simulink model "wturbines"  (R2024b)
settings: Solver=ode4  StartTime=0.0  StopTime=inf  FixedStep=0.01  RelTol=1e-3
values from neighbouring files (symbols this model uses):
  A_k = 2E6    (= 2000000)    [initialize_turbine_parameters.m]
  air_density = 1.225    [initialize_turbine_parameters.m]
  alpha_pitch_exp = 0    [initialize_turbine_parameters.m]
  B_k = 1E4    (= 10000)    [initialize_turbine_parameters.m]
  brake_torque = 28116.2    [initialize_turbine_parameters.m]
  C_k = 0    [initialize_turbine_parameters.m]
  Cp_mat = nan(numel(tsr_vec), numel(pitch_vec))    [initialize_turbine_parameters.m]
  Cp_opt = 0.482    [initialize_turbine_parameters.m]
  Ct_mat = nan(size(Cp_mat))    [initialize_turbine_parameters.m]
  ctrl_mode = 1    [initialize_turbine_parameters.m]
  cut_in_wind_speed = 3.0    (= 3)    [initialize_turbine_parameters.m]
  cut_out_wind_speed = 25.0    (= 25)    [initialize_turbine_parameters.m]
  D_k = 0    [initialize_turbine_parameters.m]
  dr_mode = Simulink.Parameter(1)    [initialize_turbine_parameters.m]
  gearbox_ratio = 1    [initialize_turbine_parameters.m]
  generator_eff = 0.954    [initialize_turbine_parameters.m]
  inertia = 1.9E6    (= 1900000)    [initialize_turbine_parameters.m]
  K_i_gen = 1e2    (= 100)    [initialize_turbine_parameters.m]
  K_i_pitch = 0    [initialize_turbine_parameters.m]
  K_i_pitch_gs = 0    [initialize_turbine_parameters.m]
  K_omega_sq = 1/2 * (tsr_opt)^-3 * air_density * pi * (rotor_diameter / 2)^5 * Cp_opt / gearbox_ratio^3    (= 69831977.2177)    [initialize_turbine_parameters.m]
  K_p_gen = 1e2    (= 100)    [initialize_turbine_parameters.m]
  K_p_pitch = 1    [initialize_turbine_parameters.m]
  K_p_pitch_gs = 0.1    [initialize_turbine_parameters.m]
  max_gen_torque = 1.15 * rated_gen_torque    (= 35686440.711)    [initialize_turbine_parameters.m]
  MIN_ROT_SPEED = 1e-3    (= 0.001)    [initialize_turbine_parameters.m]
  Nt = 9    [init.m]
  pitch_all = T{:, col_pitch}    [initialize_turbine_parameters.m]
  pitch_rate_deg = 5    [initialize_turbine_parameters.m]
  pitch_vec = sort(pitch_vec(:))    [initialize_turbine_parameters.m]
  rated_power = 22E6    (= 22000000)    [initialize_turbine_parameters.m]
  rated_rotor_speed = 6.77    [initialize_turbine_parameters.m]
  rated_rotor_speed_rads = rated_rotor_speed * (2 * pi) / 60    (= 0.70895274216)    [initialize_turbine_parameters.m]
  rated_wind_speed = 11.0    (= 11)    [initialize_turbine_parameters.m]
  ROT_EMG_MAX_TOL = 1.15    [initialize_turbine_parameters.m]
  ROT_SPEED_MIN_TRANS = min_rotor_speed_rads    (= 0.19)    [initialize_turbine_parameters.m]
  ROT_SPEED_SP_DIFF = 0.1    [initialize_turbine_parameters.m]
  rotor_radius = rotor_diameter / 2    (= 142)    [initialize_turbine_parameters.m]
  rotor_speed_all = [0, rated_rotor_speed]    [initialize_turbine_parameters.m]
  rotor_speed_init = rotor_speed_init * (2 * pi) / 60    (= 1.25663706144)    [initialize_turbine_parameters.m]
  rotor_speed_ref_mode = 1    [initialize_turbine_parameters.m]
  tsr_opt = 9.153    [initialize_turbine_parameters.m]
  tsr_vec = sort(tsr_vec(:))    [initialize_turbine_parameters.m]
  u_all = T{:, col_u}    [initialize_turbine_parameters.m]
  u_rotor_speed_all = [cut_in_wind_speed, rated_wind_speed]    [initialize_turbine_parameters.m]
  yawing_rate = 5    [initialize_turbine_parameters.m]
undefined symbols (not defined in the file or in its folder): op_mode, turbineDataBytes
libraries: simulink x24, simulink_extras x14, slpidlib x8, slrealtimeiplib x4, svdutilitieslib x2, slctrl_autotuning x2, etargetslib x2, dspstat3 x1
(part 1 of 3)
settings Model: SimulationMode=external  ExtModeEnableFloating=off  Creator=ivovanstraalen  LastModifiedBy=hackaton26
settings SolverCC: ConcurrentTasks=on  PositivePriorityOrder=on
settings DataIOCC: InspectSignalLogs=on
settings OptimizationCC: BlockReduction=off  OptimizeBlockIOStorage=off
settings DebuggingCC: SignalInfNanChecking=error  TasksWithSamePriorityMsg=none
settings HardwareCC: ProdBitPerLong=64  ProdLongLongMode=on  ProdHWDeviceType=Intel->x86-64 (Linux 64)
settings RTWCC: Description=Speedgoat Real-Time Target Machine  SystemTargetFile=speedgoat.tlc  TemplateMakefile=slrealtime_default_tmf  Toolchain=Simulink Real-Time Toolchain  BuildConfiguration=Faster Runs  CodeExecutionProfiling=on  TargetLang=C++
settings SimulinkRealTimeTargetCC: InstructionSetFMA=off  LogToMDFFile=off

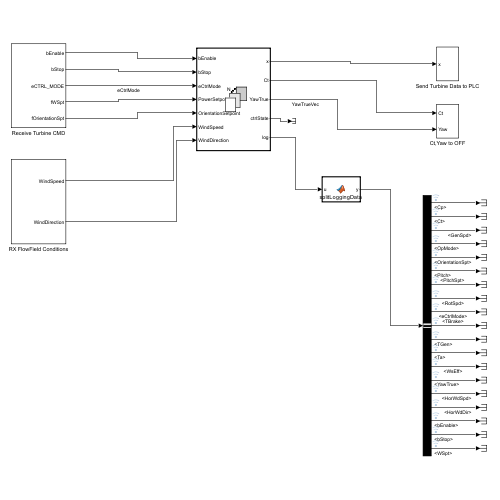
[thumbnail: Simulink's stored preview of the top-level diagram]
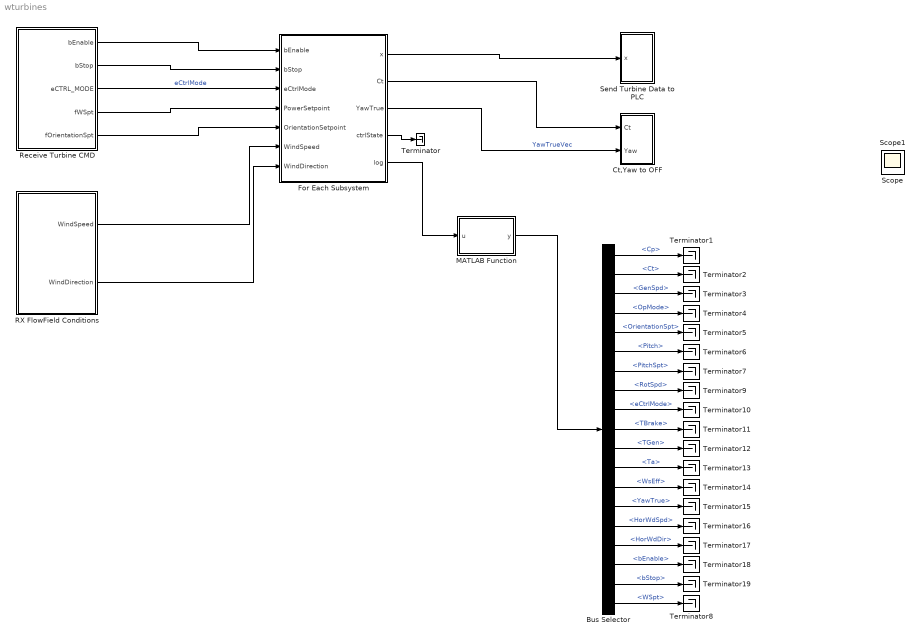
== system wturbines ==
  Bus Selector : BusSelector  OutputSignals=Cp,Ct,GenSpd,OpMode,OrientationSpt,Pitch,PitchSpt,RotSpd,eCtrlMode,TBrake,TGen,Ta,WsEff,YawTrue,HorWdSpd,HorWdDir,bEnable,bStop,WSpt
  Ct,Yaw to OFF : Subsystem
  For Each Subsystem : Subsystem  TreatAsAtomicUnit=on
  MATLAB Function : MATLAB Function  TreatAsAtomicUnit=on
  RX FlowField Conditions : Subsystem
  Receive Turbine CMD : Subsystem
  Send Turbine Data to PLC : Subsystem
  Terminator{,1..19} (20 alike) : Terminator
  Scope : Scope
  Scope1 : Scope
  wires:
  For Each Subsystem/1(x) -> Send Turbine Data to PLC/1(x)
  Receive Turbine CMD/1(bEnable) -> For Each Subsystem/1(bEnable)
  Receive Turbine CMD/4(fWSpt) -> For Each Subsystem/4(PowerSetpoint)
  Receive Turbine CMD/5(fOrientationSpt) -> For Each Subsystem/5(OrientationSetpoint)
  For Each Subsystem/2(Ct) -> Ct,Yaw to OFF/1(Ct)
  For Each Subsystem/3(YawTrue) -> Ct,Yaw to OFF/2(Yaw)  "YawTrueVec"
  RX FlowField Conditions/1(WindSpeed) -> For Each Subsystem/6(WindSpeed)
  RX FlowField Conditions/2(WindDirection) -> For Each Subsystem/7(WindDirection)
  Receive Turbine CMD/2(bStop) -> For Each Subsystem/2(bStop)
  Receive Turbine CMD/3(eCTRL_MODE) -> For Each Subsystem/3(eCtrlMode)  "eCtrlMode"
  For Each Subsystem/4(ctrlState) -> Terminator/1
  For Each Subsystem/5(log) -> MATLAB Function/1(u)
  MATLAB Function/1(y) -> Bus Selector/1
  Bus Selector/1 -> Terminator1/1  "<Cp>"
  Bus Selector/2 -> Terminator2/1  "<Ct>"
  Bus Selector/3 -> Terminator3/1  "<GenSpd>"
  Bus Selector/4 -> Terminator4/1  "<OpMode>"
  Bus Selector/5 -> Terminator5/1  "<OrientationSpt>"
  Bus Selector/6 -> Terminator6/1  "<Pitch>"
  Bus Selector/7 -> Terminator7/1  "<PitchSpt>"
  Bus Selector/8 -> Terminator9/1  "<RotSpd>"
  Bus Selector/9 -> Terminator10/1  "<eCtrlMode>"
  Bus Selector/10 -> Terminator11/1  "<TBrake>"
  Bus Selector/11 -> Terminator12/1  "<TGen>"
  Bus Selector/12 -> Terminator13/1  "<Ta>"
  Bus Selector/13 -> Terminator14/1  "<WsEff>"
  Bus Selector/14 -> Terminator15/1  "<YawTrue>"
  Bus Selector/15 -> Terminator16/1  "<HorWdSpd>"
  Bus Selector/16 -> Terminator17/1  "<HorWdDir>"
  Bus Selector/17 -> Terminator18/1  "<bEnable>"
  Bus Selector/18 -> Terminator19/1  "<bStop>"
  Bus Selector/19 -> Terminator8/1  "<WSpt>"

== system wturbines/Ct,Yaw to OFF ==
  Ct : Inport
  Yaw : Inport  Port=2
  Byte Pack1 : svdutilitieslib/Byte Pack  maskPackedDataType=uint8  datatypes={'single'}  byteAlign=1  blockPlatform=tic2000
      settings: LibrarySourceBlock=c2000lib/Target Communication/Byte Pack
  Constant1 : Constant  Value=Nt * 2*4
  Data Type Conversion : DataTypeConversion  OutDataTypeStr=single  SaturateOnIntegerOverflow=off  RndMeth=Floor
  Mux : Mux  Inputs=2
  Rate Transition : RateTransition
  UDP Send1 : slrealtimeiplib/UDP Send  useHostTargetConn=off  toAddress=pcIP  toPort=pcRXport  sampleTime=Ts_FF  enableMessage=off  ipAddress=localIP  localPort=rtsTXFFport
  wires:
  Data Type Conversion/1 -> Byte Pack1/1
  Constant1/1 -> UDP Send1/2
  Byte Pack1/1 -> UDP Send1/1
  Rate Transition/1 -> Data Type Conversion/1
  Yaw/1 -> Mux/2
  Ct/1 -> Mux/1
  Mux/1 -> Rate Transition/1

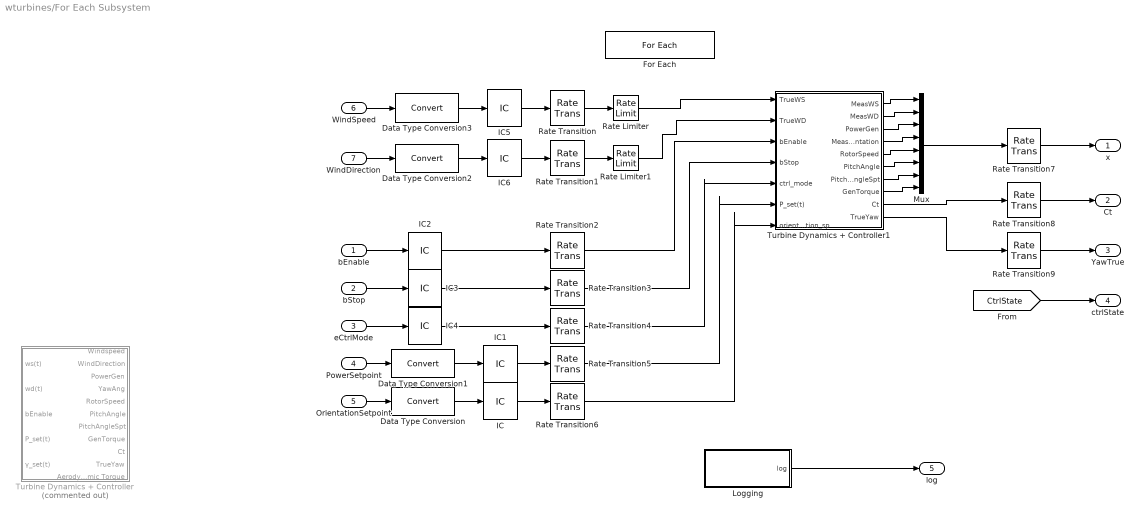
== system wturbines/For Each Subsystem ==
  bEnable : Inport  Partition=on  PartitionDimension=1  PartitionWidth=1  PartitionOffset=0
  bStop : Inport  Port=2  Partition=on  PartitionDimension=1  PartitionWidth=1  PartitionOffset=0
  eCtrlMode : Inport  Port=3  Partition=on  PartitionDimension=1  PartitionWidth=1  PartitionOffset=0
  PowerSetpoint : Inport  Port=4  Partition=on  PartitionDimension=1  PartitionWidth=1  PartitionOffset=0
  OrientationSetpoint : Inport  Port=5  Partition=on  PartitionDimension=1  PartitionWidth=1  PartitionOffset=0
  WindSpeed : Inport  Port=6  Partition=on  PartitionDimension=1  PartitionWidth=1  PartitionOffset=0
  WindDirection : Inport  Port=7  Partition=on  PartitionDimension=1  PartitionWidth=1  PartitionOffset=0
  Data Type Conversion{,1..3} (4 alike) : DataTypeConversion  SaturateOnIntegerOverflow=off  RndMeth=Floor
  For Each : ForEach  DisableCoverage=on  ShowIterationIndex=on
  IC : InitialCondition  Value=270
  IC1 : InitialCondition  Value=-1
  IC2 : InitialCondition  Value=false
  IC3 : InitialCondition  Value=false
  IC4 : InitialCondition
  IC5 : InitialCondition  Value=0
  IC6 : InitialCondition  Value=0
  Logging : Subsystem
  Mux : Mux  Inputs=8
  Rate Limiter : RateLimiter  RisingSlewLimit=inf  FallingSlewLimit=-inf  SampleTimeMode=inherited
  Rate Limiter1 : RateLimiter  RisingSlewLimit=inf  FallingSlewLimit=-inf  SampleTimeMode=inherited
  Rate Transition{,1..9} (10 alike) : RateTransition
  Turbine Dynamics + Controller : Subsystem  Commented=on
  Turbine Dynamics + Controller1 : Subsystem
  x : Outport  ConcatenationDimension=1
  Ct : Outport  Port=2  ConcatenationDimension=1
  YawTrue : Outport  Port=3  ConcatenationDimension=1
  ctrlState : Outport  Port=4  ConcatenationDimension=1
  log : Outport  Port=5  ConcatenationDimension=1
  wires:
  Turbine Dynamics + Controller1/1(MeasWS) -> Mux/1
  Turbine Dynamics + Controller1/2(MeasWD) -> Mux/2
  Turbine Dynamics + Controller1/3(PowerGen) -> Mux/3
  Turbine Dynamics + Controller1/4(MeasOrientation) -> Mux/4
  Turbine Dynamics + Controller1/5(RotorSpeed) -> Mux/5
  Turbine Dynamics + Controller1/6(PitchAngle) -> Mux/6
  Turbine Dynamics + Controller1/7(PitchAngleSpt) -> Mux/7
  Turbine Dynamics + Controller1/8(GenTorque) -> Mux/8
  Mux/1 -> Rate Transition7/1
  bEnable/1 -> IC2/1
  Data Type Conversion1/1 -> IC1/1
  Data Type Conversion/1 -> IC/1
  OrientationSetpoint/1 -> Data Type Conversion/1
  PowerSetpoint/1 -> Data Type Conversion1/1
  IC/1 -> Rate Transition6/1
  IC1/1 -> Rate Transition5/1
  IC2/1 -> Rate Transition2/1
  Turbine Dynamics + Controller1/9(Ct) -> Rate Transition8/1
  Turbine Dynamics + Controller1/10(TrueYaw) -> Rate Transition9/1
  bStop/1 -> IC3/1
  eCtrlMode/1 -> IC4/1
  IC3/1 -> Rate Transition3/1
  IC4/1 -> Rate Transition4/1
  WindSpeed/1 -> Data Type Conversion3/1
  WindDirection/1 -> Data Type Conversion2/1
  Data Type Conversion2/1 -> IC6/1
  Data Type Conversion3/1 -> IC5/1
  IC5/1 -> Rate Transition/1
  IC6/1 -> Rate Transition1/1
  Rate Transition2/1 -> Turbine Dynamics + Controller1/3(bEnable)
  Rate Transition3/1 -> Turbine Dynamics + Controller1/4(bStop)
  Rate Transition4/1 -> Turbine Dynamics + Controller1/5(ctrl_mode)
  Rate Transition5/1 -> Turbine Dynamics + Controller1/6(P_set(t))
  Rate Transition6/1 -> Turbine Dynamics + Controller1/7(orientation_sp)
  Rate Transition7/1 -> x/1
  Rate Transition8/1 -> Ct/1
  Rate Transition9/1 -> YawTrue/1
  [CtrlState] -> ctrlState/1
  Rate Transition1/1 -> Rate Limiter1/1
  Rate Transition/1 -> Rate Limiter/1
  Rate Limiter/1 -> Turbine Dynamics + Controller1/1(TrueWS)
  Rate Limiter1/1 -> Turbine Dynamics + Controller1/2(TrueWD)
  Logging/1(log) -> log/1

== system wturbines/RX FlowField Conditions ==
  Compare To Constant : simulink/Logic and Bit Operations/Compare To Constant  relop=>  const=0  OutDataTypeStr=boolean
  Enabled Subsystem : Subsystem  TreatAsAtomicUnit=on
  Rate Transition1 : RateTransition
  Rate Transition2 : RateTransition
  UDP Receive : slrealtimeiplib/UDP Receive  useHostTargetConn=off  ipAddress=localIP  localPort=rtsRXFFport  rcvWidth=2*4*Nt  rcvFmAny=off  fmAddress=pcIP  sampleTime=0.1  enableMessage=off  maxPackets=1
  WindSpeed : Outport
  WindDirection : Outport  Port=2
  wires:
  UDP Receive/2 -> Compare To Constant/1
  Enabled Subsystem/1(WindSpeed) -> Rate Transition1/1
  Rate Transition2/1 -> WindDirection/1
  Rate Transition1/1 -> WindSpeed/1
  UDP Receive/1 -> Enabled Subsystem/1(In1)
  Compare To Constant/1 -> Enabled Subsystem/Enable
  Enabled Subsystem/2(Wind Direction) -> Rate Transition2/1

== system wturbines/Receive Turbine CMD ==
  Compare To Constant : simulink/Logic and Bit Operations/Compare To Constant  relop=>  const=0  OutDataTypeStr=boolean
  Enabled Subsystem : Subsystem  TreatAsAtomicUnit=on
  Rate Transition{,1..4} (5 alike) : RateTransition
  UDP Receive : slrealtimeiplib/UDP Receive  useHostTargetConn=off  ipAddress=localIP  localPort=10000  rcvWidth=(1+1+1+4+4)*Nt  rcvFmAny=off  fmAddress=plcIP  sampleTime=0.1  enableMessage=off  maxPackets=1
  bEnable : Outport
  bStop : Outport  Port=2
  eCTRL_MODE : Outport  Port=3
  fWSpt : Outport  Port=4
  fOrientationSpt : Outport  Port=5
  wires:
  Enabled Subsystem/1(bEnable) -> Rate Transition/1
  UDP Receive/2 -> Compare To Constant/1
  Enabled Subsystem/4(fPowerSpt) -> Rate Transition1/1
  Rate Transition2/1 -> fOrientationSpt/1
  Rate Transition1/1 -> fWSpt/1
  UDP Receive/1 -> Enabled Subsystem/1(In1)
  Rate Transition/1 -> bEnable/1
  Compare To Constant/1 -> Enabled Subsystem/Enable
  Enabled Subsystem/5(fYawSpt) -> Rate Transition2/1
  Rate Transition3/1 -> bStop/1
  Enabled Subsystem/3(eCTRL_MODE) -> Rate Transition4/1
  Rate Transition4/1 -> eCTRL_MODE/1
  Enabled Subsystem/2(bStop) -> Rate Transition3/1

== system wturbines/Send Turbine Data to PLC ==
  x : Inport
  Byte Pack1 : svdutilitieslib/Byte Pack  maskPackedDataType=uint8  datatypes={'single'}  byteAlign=1  blockPlatform=tic2000
      settings: LibrarySourceBlock=c2000lib/Target Communication/Byte Pack
  Constant1 : Constant  Value=Nt * turbineDataBytes
  Data Type Conversion : DataTypeConversion  OutDataTypeStr=single  SaturateOnIntegerOverflow=off  RndMeth=Floor
  Rate Transition : RateTransition
  UDP Send1 : slrealtimeiplib/UDP Send  useHostTargetConn=off  toAddress=plcIP  toPort=plcRXport  sampleTime=Ts_IEC  enableMessage=off  ipAddress=localIP  localPort=11000
  wires:
  Data Type Conversion/1 -> Byte Pack1/1
  Constant1/1 -> UDP Send1/2
  Byte Pack1/1 -> UDP Send1/1
  Rate Transition/1 -> Data Type Conversion/1
  x/1 -> Rate Transition/1

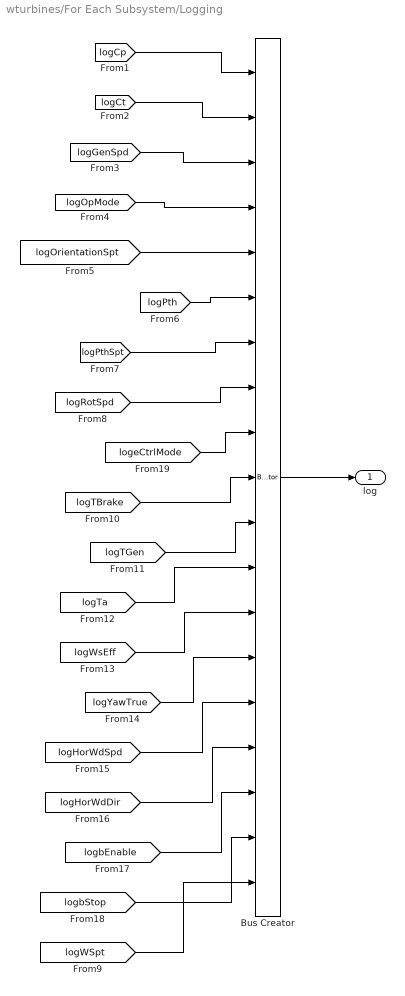
== system wturbines/For Each Subsystem/Logging ==
  Bus Creator : BusCreator  Inputs=19  OutDataTypeStr=Bus: loggingData  NonVirtualBus=on
  log : Outport
  wires:
  [logCp] -> Bus Creator/1
  [logCt] -> Bus Creator/2
  [logGenSpd] -> Bus Creator/3
  [logOpMode] -> Bus Creator/4
  [logOrientationSpt] -> Bus Creator/5
  [logPth] -> Bus Creator/6
  [logPthSpt] -> Bus Creator/7
  [logRotSpd] -> Bus Creator/8
  [logeCtrlMode] -> Bus Creator/9
  [logTBrake] -> Bus Creator/10
  [logTGen] -> Bus Creator/11
  [logTa] -> Bus Creator/12
  [logWsEff] -> Bus Creator/13
  [logYawTrue] -> Bus Creator/14
  [logHorWdSpd] -> Bus Creator/15
  [logHorWdDir] -> Bus Creator/16
  [logbEnable] -> Bus Creator/17
  [logbStop] -> Bus Creator/18
  Bus Creator/1 -> log/1
  [logWSpt] -> Bus Creator/19

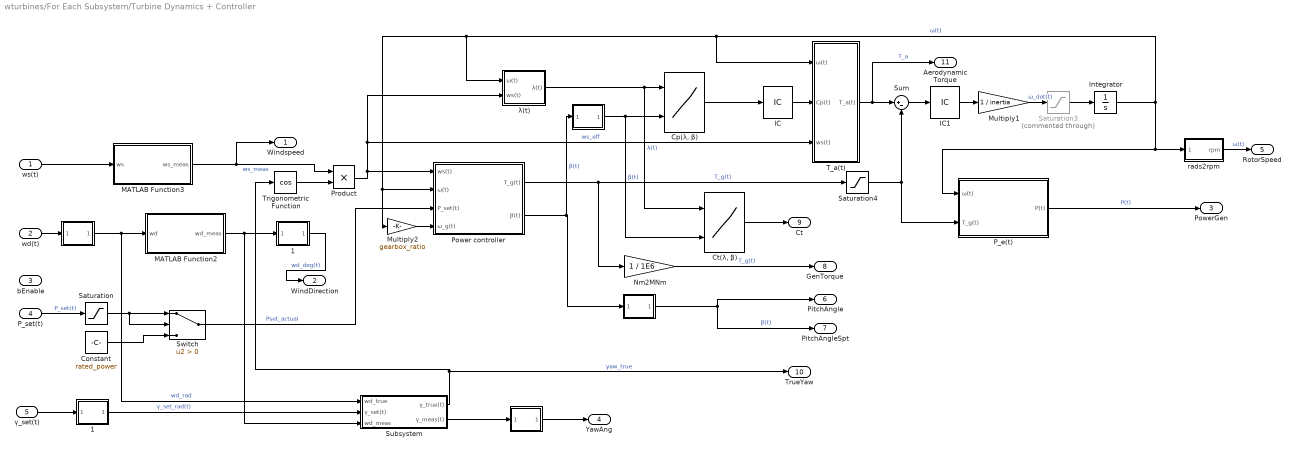
== system wturbines/For Each Subsystem/Turbine Dynamics + Controller ==
  ws(t) : Inport
  wd(t) : Inport  Port=2
  bEnable : Inport  Port=3
  P_set(t) : Inport  Port=4
  γ_set(t) : Inport  Port=5
  " " : Subsystem
  "  " : Subsystem
  "   " : Subsystem
  "     " : Subsystem
  "     1" : Subsystem
  "   1" : Subsystem
  Constant : Constant  Value=rated_power
  "Cp(λ, β)" : Lookup_n-D  BreakpointsForDimension1=tsr_vec  BreakpointsForDimension2=pitch_vec  Table=Cp_mat  InterpMethod=Cubic spline  ExtrapMethod=Clip  DiagnosticForOutOfRangeInput=Error  InternalRulePriority=Speed  RndMeth=Simplest
      settings: InputPortMap=u0,u1
  "Ct(λ, β)" : Lookup_n-D  BreakpointsForDimension1=tsr_vec  BreakpointsForDimension2=pitch_vec  Table=Ct_mat  InterpMethod=Cubic spline  ExtrapMethod=Clip  DiagnosticForOutOfRangeInput=Error  InternalRulePriority=Speed  RndMeth=Simplest
      settings: InputPortMap=u0,u1
  IC : InitialCondition  Value=0.6
  IC1 : InitialCondition  Value=0
  Integrator : Integrator  InitialCondition=rotor_speed_init  LimitOutput=on  LowerSaturationLimit=0
  MATLAB Function2 : MATLAB Function  TreatAsAtomicUnit=on
  MATLAB Function3 : MATLAB Function  TreatAsAtomicUnit=on
  Multiply1 : Gain  Gain=1 / inertia
  Multiply2 : Gain  Gain=gearbox_ratio
  Nm2MNm : Gain  Gain=1 / 1E6
  P_e(t) : Subsystem
  Power controller : Subsystem
  Product : Product
  Saturation : Saturate  UpperLimit=rated_power  LowerLimit=0
  Saturation3 : Saturate  Commented=through  UpperLimit=inf  LowerLimit=-inf
  Saturation4 : Saturate  UpperLimit=inf  LowerLimit=0
  Subsystem : Subsystem
  Sum : Sum  Inputs=|+-
  Switch : Switch  Criteria=u2 > Threshold  SaturateOnIntegerOverflow=off  InputSameDT=off
  T_a(t) : Subsystem
  Trigonometric Function : Trigonometry  Operator=cos
  rads2rpm : Subsystem
  λ(t) : Subsystem
  Windspeed : Outport
  WindDirection : Outport  Port=2
  PowerGen : Outport  Port=3
  YawAng : Outport  Port=4
  RotorSpeed : Outport  Port=5
  PitchAngle : Outport  Port=6
  PitchAngleSpt : Outport  Port=7
  GenTorque : Outport  Port=8
  Ct : Outport  Port=9
  TrueYaw : Outport  Port=10
  Aerodynamic Torque : Outport  Port=11
  wires:
  P_e(t)/1(P(t)) -> PowerGen/1  "P(t)"
  Power controller/1(T_g(t)) -> Saturation4/1, Nm2MNm/1  "T_g(t)"
  λ(t)/1(λ(t)) -> "Cp(λ, β)"/1, "Ct(λ, β)"/1  "λ(t)"
  P_set(t)/1 -> Saturation/1  "P_set(t)"
  Multiply2/1 -> Power controller/4(ω_g(t))
  rads2rpm/1(rpm) -> RotorSpeed/1  "ω(t)"
  Sum/1 -> IC1/1
  Integrator/1 -> λ(t)/1(ω(t)), Multiply2/1, Power controller/2(ω(t)), T_a(t)/1(ω(t)), P_e(t)/1(ω(t)), rads2rpm/1(rad/s)  "ω(t)"
  Multiply1/1 -> Saturation3/1  "ω_dot(t)"
  "  "/1(deg) -> "Cp(λ, β)"/2, "Ct(λ, β)"/2  "β(t)"
  "   "/1(deg) -> PitchAngleSpt/1, PitchAngle/1  "β(t)"
  Power controller/2(β(t)) -> "  "/1(rad), "   "/1(rad)  "β(t)"
  Product/1 -> Power controller/1(ws(t)), λ(t)/2(ws(t)), T_a(t)/3(ws(t))  "ws_eff"
  T_a(t)/1(T_a(t)) -> Aerodynamic Torque/1, Sum/1  "T_a"
  Nm2MNm/1 -> GenTorque/1  "T_g(t)"
  Saturation/1 -> Switch/1, Switch/2
  wd(t)/1 -> "     "/1(deg)
  "     "/1(rad) -> MATLAB Function2/1(wd), Subsystem/1(wd_true)  "wd_rad"
  Trigonometric Function/1 -> Product/2
  ws(t)/1 -> MATLAB Function3/1(ws)
  Constant/1 -> Switch/3
  Switch/1 -> Power controller/3(P_set(t))  "Pset_actual"
  MATLAB Function2/1(wd_meas) -> Subsystem/3(wd_meas), "   1"/1(rad)
  MATLAB Function3/1(ws_meas) -> Windspeed/1, Product/1  "ws_meas"
  γ_set(t)/1 -> "     1"/1(deg)
  Subsystem/1(γ_true(t)) -> Trigonometric Function/1, TrueYaw/1  "yaw_true"
  " "/1(deg) -> YawAng/1
  Subsystem/2(γ_meas(t)) -> " "/1(rad)
  "     1"/1(rad) -> Subsystem/2(γ_set(t))  "γ_set_rad(t)"
  "   1"/1(deg) -> WindDirection/1  "wd_deg(t)"
  IC/1 -> T_a(t)/2(Cp(t))
  "Cp(λ, β)"/1 -> IC/1
  IC1/1 -> Multiply1/1
  "Ct(λ, β)"/1 -> Ct/1
  Saturation3/1 -> Integrator/1
  Saturation4/1 -> Sum/2, P_e(t)/2(T_g(t))

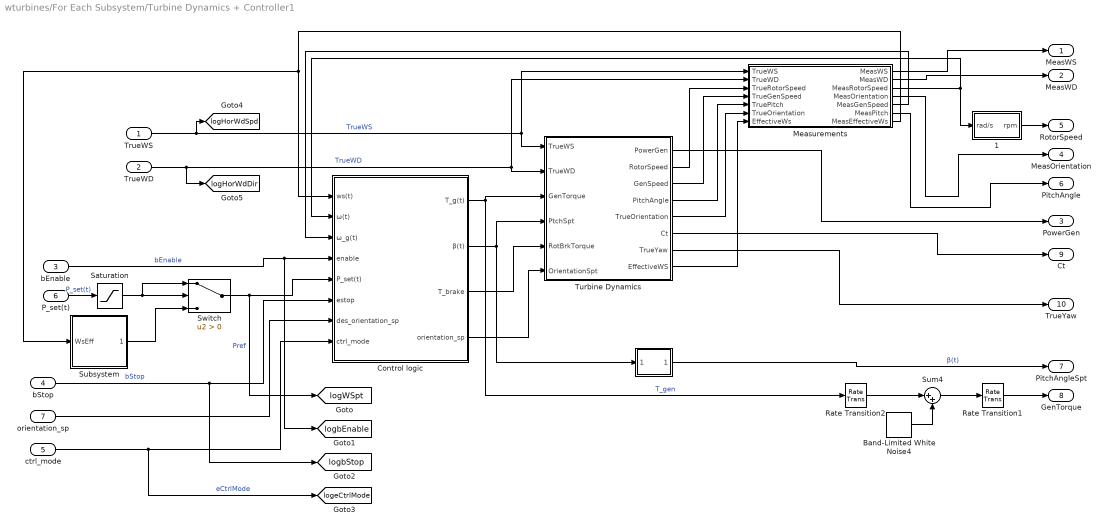
== system wturbines/For Each Subsystem/Turbine Dynamics + Controller1 ==
  TrueWS : Inport
  TrueWD : Inport  Port=2
  bEnable : Inport  Port=3
  bStop : Inport  Port=4
  ctrl_mode : Inport  Port=5
  P_set(t) : Inport  Port=6
  orientation_sp : Inport  Port=7
  "  " : Subsystem
  "  1" : Subsystem
  Band-Limited White Noise4 : simulink/Sources/Band-Limited White Noise  Cov=[.001]  Ts=0.1  seed=[23341]
  Control logic : Subsystem
  Measurements : Subsystem
  Rate Transition1 : RateTransition
  Rate Transition2 : RateTransition
  Saturation : Saturate  UpperLimit=rated_power  LowerLimit=0
  Subsystem : Subsystem
  Sum4 : Sum  Inputs=|++
  Switch : Switch  Criteria=u2 > Threshold  SaturateOnIntegerOverflow=off  InputSameDT=off
  Turbine Dynamics : Subsystem
  MeasWS : Outport
  MeasWD : Outport  Port=2
  PowerGen : Outport  Port=3
  MeasOrientation : Outport  Port=4
  RotorSpeed : Outport  Port=5
  PitchAngle : Outport  Port=6
  PitchAngleSpt : Outport  Port=7
  GenTorque : Outport  Port=8
  Ct : Outport  Port=9
  TrueYaw : Outport  Port=10
  tag scope: logHorWdDir=global, logHorWdSpd=global, logWSpt=global, logbEnable=global, logbStop=global, logeCtrlMode=global
  wires:
  Control logic/1(T_g(t)) -> Rate Transition2/1, Turbine Dynamics/3(GenTorque)  "T_gen"
  Control logic/2(β(t)) -> Turbine Dynamics/4(PtchSpt), "  "/1(rad)
  Control logic/3(T_brake) -> Turbine Dynamics/5(RotBrkTorque)
  Turbine Dynamics/4(PitchAngle) -> Measurements/5(TruePitch)
  Turbine Dynamics/2(RotorSpeed) -> Measurements/3(TrueRotorSpeed)
  TrueWD/1 -> [logHorWdDir], Measurements/2(TrueWD), Turbine Dynamics/2(TrueWD)  "TrueWD"
  Measurements/1(MeasWS) -> MeasWS/1
  Measurements/2(MeasWD) -> MeasWD/1
  Measurements/4(MeasOrientation) -> MeasOrientation/1
  Measurements/3(MeasRotorSpeed) -> "  1"/1(rad/s), Control logic/2(ω(t))
  Measurements/6(MeasPitch) -> PitchAngle/1
  Turbine Dynamics/1(PowerGen) -> PowerGen/1
  Turbine Dynamics/3(GenSpeed) -> Measurements/4(TrueGenSpeed)
  Measurements/5(MeasGenSpeed) -> Control logic/3(ω_g(t))
  bEnable/1 -> [logbEnable], Control logic/4(enable)  "bEnable"
  Switch/1 -> [logWSpt], Control logic/5(P_set(t))  "Pref"
  TrueWS/1 -> [logHorWdSpd], Turbine Dynamics/1(TrueWS), Measurements/1(TrueWS)  "TrueWS"
  Turbine Dynamics/7(TrueYaw) -> TrueYaw/1
  Turbine Dynamics/5(TrueOrientation) -> Measurements/6(TrueOrientation)
  Turbine Dynamics/6(Ct) -> Ct/1
  orientation_sp/1 -> Control logic/7(des_orientation_sp)
  bStop/1 -> [logbStop], Control logic/6(estop)  "bStop"
  Control logic/4(orientation_sp) -> Turbine Dynamics/6(OrientationSpt)
  ctrl_mode/1 -> [logeCtrlMode], Control logic/8(ctrl_mode)  "eCtrlMode"
  Saturation/1 -> Switch/1, Switch/2
  Subsystem/1(P_avail) -> Switch/3
  P_set(t)/1 -> Saturation/1  "P_set(t)"
  "  "/1(deg) -> PitchAngleSpt/1  "β(t)"
  "  1"/1(rpm) -> RotorSpeed/1
  Measurements/7(MeasEffectiveWs) -> Subsystem/1(WsEff), Control logic/1(ws(t))
  Turbine Dynamics/8(EffectiveWS) -> Measurements/7(EffectiveWs)
  Sum4/1 -> Rate Transition1/1
  Band-Limited White Noise4/1 -> Sum4/2
  Rate Transition2/1 -> Sum4/1
  Rate Transition1/1 -> GenTorque/1

== system wturbines/RX FlowField Conditions/Enabled Subsystem ==
  In1 : Inport
  Enable : EnablePort
  Byte Unpack : etargetslib/Byte Unpack  dimensions={[Nt], [Nt]}  datatypes={ 'single', 'single'}  byteAlign=1
      settings: LibrarySourceBlock=embeddedtargetslib/Host Communication/Byte Unpack
  Unit Delay : UnitDelay  InitialCondition=zeros(Nt,1)  SampleTime=-1  HasFrameUpgradeWarning=on
  Unit Delay1 : UnitDelay  InitialCondition=zeros(Nt,1)  SampleTime=-1  HasFrameUpgradeWarning=on
  ZoH nan filter1 : MATLAB Function  TreatAsAtomicUnit=on
  ZoH nan filter2 : MATLAB Function  TreatAsAtomicUnit=on
  WindSpeed : Outport
  Wind Direction : Outport  Port=2
  wires:
  Byte Unpack/1 -> ZoH nan filter1/1(w)
  In1/1 -> Byte Unpack/1
  ZoH nan filter1/1(w_filtered) -> Unit Delay/1, WindSpeed/1
  Unit Delay/1 -> ZoH nan filter1/2(w_saved)
  Unit Delay1/1 -> ZoH nan filter2/2(w_saved)
  Byte Unpack/2 -> ZoH nan filter2/1(w)
  ZoH nan filter2/1(w_filtered) -> Wind Direction/1, Unit Delay1/1

== system wturbines/Receive Turbine CMD/Enabled Subsystem ==
  In1 : Inport
  Enable : EnablePort
  Byte Unpack : etargetslib/Byte Unpack  dimensions={[Nt], [Nt], [Nt], [Nt], [Nt]}  datatypes={'boolean', 'boolean', 'uint8', 'single', 'single'}  byteAlign=1
      settings: LibrarySourceBlock=embeddedtargetslib/Host Communication/Byte Unpack
  Zero-Order Hold{,1..4} (5 alike) : ZeroOrderHold  SampleTime=-1
  bEnable : Outport
  bStop : Outport  Port=2
  eCTRL_MODE : Outport  Port=3
  fPowerSpt : Outport  Port=4
  fYawSpt : Outport  Port=5
  wires:
  Byte Unpack/2 -> Zero-Order Hold1/1
  Byte Unpack/1 -> Zero-Order Hold/1
  Zero-Order Hold1/1 -> bStop/1
  Byte Unpack/3 -> Zero-Order Hold2/1
  Zero-Order Hold/1 -> bEnable/1
  In1/1 -> Byte Unpack/1
  Zero-Order Hold2/1 -> eCTRL_MODE/1
  Zero-Order Hold3/1 -> fPowerSpt/1
  Zero-Order Hold4/1 -> fYawSpt/1
  Byte Unpack/4 -> Zero-Order Hold3/1
  Byte Unpack/5 -> Zero-Order Hold4/1

== system wturbines/For Each Subsystem/Turbine Dynamics + Controller/  ==
  rad : Inport
  Radians to Degrees : simulink_extras/Transformations/Radians to Degrees
  deg : Outport
  wires:
  Radians to Degrees/1 -> deg/1
  rad/1 -> Radians to Degrees/1

== system wturbines/For Each Subsystem/Turbine Dynamics + Controller/   ==
  rad : Inport
  Radians to Degrees : simulink_extras/Transformations/Radians to Degrees
  deg : Outport
  wires:
  Radians to Degrees/1 -> deg/1
  rad/1 -> Radians to Degrees/1

== system wturbines/For Each Subsystem/Turbine Dynamics + Controller/    ==
  rad : Inport
  Radians to Degrees : simulink_extras/Transformations/Radians to Degrees
  deg : Outport
  wires:
  Radians to Degrees/1 -> deg/1
  rad/1 -> Radians to Degrees/1

== system wturbines/For Each Subsystem/Turbine Dynamics + Controller/      ==
  deg : Inport
  Degrees to Radians : simulink_extras/Transformations/Degrees to Radians
  rad : Outport
  wires:
  Degrees to Radians/1 -> rad/1
  deg/1 -> Degrees to Radians/1

== system wturbines/For Each Subsystem/Turbine Dynamics + Controller/     1 ==
  deg : Inport
  Degrees to Radians : simulink_extras/Transformations/Degrees to Radians
  rad : Outport
  wires:
  Degrees to Radians/1 -> rad/1
  deg/1 -> Degrees to Radians/1

== system wturbines/For Each Subsystem/Turbine Dynamics + Controller/   1 ==
  rad : Inport
  Radians to Degrees : simulink_extras/Transformations/Radians to Degrees
  deg : Outport
  wires:
  Radians to Degrees/1 -> deg/1
  rad/1 -> Radians to Degrees/1

== system wturbines/For Each Subsystem/Turbine Dynamics + Controller/P_e(t) ==
  ω(t) : Inport
  T_g(t) : Inport  Port=2
  Multiply : Gain  Gain=generator_eff
  Product : Product
  P(t) : Outport
  wires:
  Product/1 -> Multiply/1
  Multiply/1 -> P(t)/1
  T_g(t)/1 -> Product/2
  ω(t)/1 -> Product/1

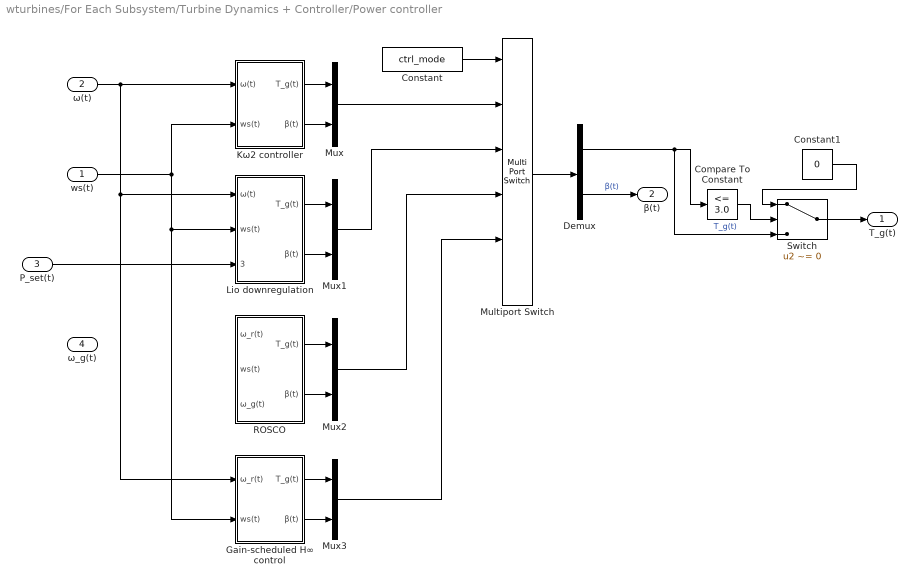
== system wturbines/For Each Subsystem/Turbine Dynamics + Controller/Power controller ==
  ws(t) : Inport
  ω(t) : Inport  Port=2
  P_set(t) : Inport  Port=3
  ω_g(t) : Inport  Port=4
  Compare To Constant : simulink/Logic and Bit Operations/Compare To Constant  relop=<=  const=3.0  OutDataTypeStr=boolean
  Constant : Constant  Value=ctrl_mode
  Constant1 : Constant  Value=0
  Demux : Demux  Outputs=2
  "Gain-scheduled H∞ control " : Subsystem
  Kω2 controller : Subsystem
  Lio downregulation : Subsystem
  Multiport Switch : MultiPortSwitch  Inputs=4  DataPortForDefault=Additional data port  SaturateOnIntegerOverflow=off  InputSameDT=off
  Mux{,1..3} (4 alike) : Mux  Inputs=2
  ROSCO : Subsystem
  Switch : Switch  Criteria=u2 ~= 0  SaturateOnIntegerOverflow=off  InputSameDT=off
  T_g(t) : Outport
  β(t) : Outport  Port=2
  wires:
  Mux3/1 -> Multiport Switch/5
  Mux2/1 -> Multiport Switch/4
  "Gain-scheduled H∞ control "/2(β(t)) -> Mux3/2
  "Gain-scheduled H∞ control "/1(T_g(t)) -> Mux3/1
  ROSCO/1(T_g(t)) -> Mux2/1
  ROSCO/2(β(t)) -> Mux2/2
  Mux1/1 -> Multiport Switch/3
  Mux/1 -> Multiport Switch/2
  Lio downregulation/2(β(t)) -> Mux1/2
  Lio downregulation/1(T_g(t)) -> Mux1/1
  Demux/2 -> β(t)/1  "β(t)"
  Demux/1 -> Switch/3, Compare To Constant/1  "T_g(t)"
  Multiport Switch/1 -> Demux/1
  Constant/1 -> Multiport Switch/1
  P_set(t)/1 -> Lio downregulation/3(P_set(t))
  ws(t)/1 -> "Gain-scheduled H∞ control "/2(ws(t)), Lio downregulation/2(ws(t)), Kω2 controller/2(ws(t))
  ω(t)/1 -> Kω2 controller/1(ω(t)), Lio downregulation/1(ω(t)), "Gain-scheduled H∞ control "/1(ω_r(t))
  Kω2 controller/2(β(t)) -> Mux/2
  Kω2 controller/1(T_g(t)) -> Mux/1
  Compare To Constant/1 -> Switch/2
  Constant1/1 -> Switch/1
  Switch/1 -> T_g(t)/1

== system wturbines/For Each Subsystem/Turbine Dynamics + Controller/Subsystem ==
  wd_true : Inport
  γ_set(t) : Inport  Port=2
  wd_meas : Inport  Port=3
  Meas Yaw Offset : MATLAB Function  TreatAsAtomicUnit=on
  Orientation Setpoint Calculation : MATLAB Function  TreatAsAtomicUnit=on
  Scope : Scope
  True Yaw Offset : MATLAB Function  TreatAsAtomicUnit=on
  Yaw controller : Subsystem
  γ_true(t) : Outport
  γ_meas(t) : Outport  Port=2
  wires:
  True Yaw Offset/1(yaw) -> γ_true(t)/1  "γ_rad(t)"
  γ_set(t)/1 -> Orientation Setpoint Calculation/2(yaw_offset)  "γ_set_rad(t)"
  Orientation Setpoint Calculation/1(orientation) -> Scope/1, Yaw controller/1(orientation_set(t))  "orientation_sp"
  wd_true/1 -> True Yaw Offset/1(wind_dir)
  Yaw controller/1(orientation(t)) -> Meas Yaw Offset/2(orientation), True Yaw Offset/2(orientation)  "orientation(t)"
  wd_meas/1 -> Orientation Setpoint Calculation/1(wind_dir), Meas Yaw Offset/1(wind_dir)
  Meas Yaw Offset/1(yaw) -> γ_meas(t)/1  "γ_rad(t)"

== system wturbines/For Each Subsystem/Turbine Dynamics + Controller/T_a(t) ==
  ω(t) : Inport
  Cp(t) : Inport  Port=2
  ws(t) : Inport  Port=3
  Constant4 : Constant  Value=1/2
  Constant5 : Constant  Value=air_density
  Constant6 : Constant  Value=pi
  Constant7 : Constant  Value=rotor_radius
  Constant8 : Constant  Value=3
  Power : Math  Operator=pow
  Product : Product  Inputs=7
  Square : Math  Operator=square
  T_a(t) : Outport
  wires:
  Cp(t)/1 -> Product/4
  Constant7/1 -> Square/1
  Constant8/1 -> Power/2
  Power/1 -> Product/7
  Constant4/1 -> Product/2
  Constant5/1 -> Product/3
  ws(t)/1 -> Power/1
  Constant6/1 -> Product/6
  Square/1 -> Product/5
  Product/1 -> T_a(t)/1  "T_a(t)"
  ω(t)/1 -> Product/1

== system wturbines/For Each Subsystem/Turbine Dynamics + Controller/rads2rpm ==
  rad/s : Inport
  Multiply : Gain  Gain=1 / (2 * pi)
  Multiply1 : Gain  Gain=60
  rpm : Outport
  wires:
  Multiply/1 -> Multiply1/1
  rad/s/1 -> Multiply/1
  Multiply1/1 -> rpm/1

== system wturbines/For Each Subsystem/Turbine Dynamics + Controller/λ(t) ==
  ω(t) : Inport
  ws(t) : Inport  Port=2
  Constant : Constant  Value=rotor_radius
  Divide : Product  Inputs=*/
  Product : Product
  λ(t) : Outport
  wires:
  Constant/1 -> Product/2
  Divide/1 -> λ(t)/1  "λ(t)"
  ω(t)/1 -> Product/1
  Product/1 -> Divide/1
  ws(t)/1 -> Divide/2

== system wturbines/For Each Subsystem/Turbine Dynamics + Controller1/   ==
  rad : Inport
  Radians to Degrees : simulink_extras/Transformations/Radians to Degrees
  deg : Outport
  wires:
  rad/1 -> Radians to Degrees/1
  Radians to Degrees/1 -> deg/1

== system wturbines/For Each Subsystem/Turbine Dynamics + Controller1/  1 ==
  rad/s : Inport
  Gain : Gain  Gain=60/(2*pi)
  rpm : Outport
  wires:
  rad/s/1 -> Gain/1
  Gain/1 -> rpm/1

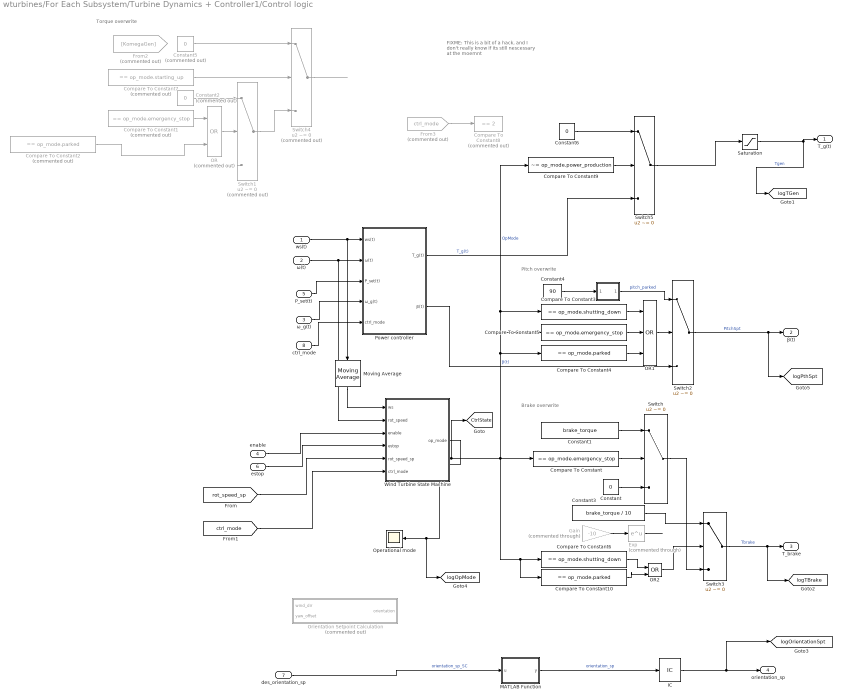
== system wturbines/For Each Subsystem/Turbine Dynamics + Controller1/Control logic ==
  note: Brake overwrite
  note: Pitch overwrite
  note: FIXME: This is a bit of a hack, and I don't really know if its still nescessary at the moemnt
  note: Torque overwrite
  ws(t) : Inport
  ω(t) : Inport  Port=2
  ω_g(t) : Inport  Port=3
  enable : Inport  Port=4
  P_set(t) : Inport  Port=5
  estop : Inport  Port=6
  des_orientation_sp : Inport  Port=7
  ctrl_mode : Inport  Port=8
  "     " : Subsystem
  Compare To Constant : simulink/Logic and Bit Operations/Compare To Constant  relop===  const=op_mode.emergency_stop  OutDataTypeStr=boolean
  Compare To Constant1 : simulink/Logic and Bit Operations/Compare To Constant  Commented=on  relop===  const=op_mode.emergency_stop  OutDataTypeStr=boolean
  Compare To Constant10 : simulink/Logic and Bit Operations/Compare To Constant  relop===  const=op_mode.parked  OutDataTypeStr=boolean
  Compare To Constant2 : simulink/Logic and Bit Operations/Compare To Constant  Commented=on  relop===  const=op_mode.parked  OutDataTypeStr=boolean
  Compare To Constant3 : simulink/Logic and Bit Operations/Compare To Constant  relop===  const=op_mode.shutting_down  OutDataTypeStr=boolean
  Compare To Constant4 : simulink/Logic and Bit Operations/Compare To Constant  relop===  const=op_mode.parked  OutDataTypeStr=boolean
  Compare To Constant5 : simulink/Logic and Bit Operations/Compare To Constant  relop===  const=op_mode.emergency_stop  OutDataTypeStr=boolean
  Compare To Constant6 : simulink/Logic and Bit Operations/Compare To Constant  relop===  const=op_mode.shutting_down  OutDataTypeStr=boolean
  Compare To Constant7 : simulink/Logic and Bit Operations/Compare To Constant  Commented=on  relop===  const=op_mode.starting_up  OutDataTypeStr=boolean
  Compare To Constant8 : simulink/Logic and Bit Operations/Compare To Constant  Commented=on  relop===  const=2  OutDataTypeStr=boolean
  Compare To Constant9 : simulink/Logic and Bit Operations/Compare To Constant  relop=~=  const=op_mode.power_production  OutDataTypeStr=boolean
  Constant : Constant  Value=0
  Constant1 : Constant  Value=brake_torque
  Constant2 : Constant  Commented=on  Value=0
  Constant3 : Constant  Value=brake_torque / 10
  Constant4 : Constant  Value=90
  Constant5 : Constant  Commented=on  Value=0
  Constant6 : Constant  Value=0
  Exp : Math  Commented=through
  From2 : From  Commented=on  GotoTag=KomegaGen
  From3 : From  Commented=on  GotoTag=ctrl_mode  TagVisibility=global
  Gain : Gain  Commented=through  Gain=-10
  IC : InitialCondition  Value=270
  MATLAB Function : MATLAB Function  TreatAsAtomicUnit=on
  Moving Average : dspstat3/Moving Average  Method=Exponential weighting  ForgettingFactorPort=off  SpecifyWindowLength=on  WindowLength=20  OverlapLength=3  AllowArbitraryInputLength=off  ForgettingFactor=0.95  SimulateUsing=Interpreted execution
  OR : Logic  Commented=on  Operator=OR  IconShape=distinctive  AllPortsSameDT=off  OutDataTypeStr=boolean
  OR1 : Logic  Operator=OR  Inputs=3  IconShape=distinctive  AllPortsSameDT=off  OutDataTypeStr=boolean
  OR2 : Logic  Operator=OR  IconShape=distinctive  AllPortsSameDT=off  OutDataTypeStr=boolean
  Operational mode : Scope
  Orientation Setpoint Calculation : MATLAB Function  Commented=on  TreatAsAtomicUnit=on
  Power controller : Subsystem
  Saturation : Saturate  UpperLimit=max_gen_torque  LowerLimit=0
  Switch{,2..3,5} (4 alike) : Switch  Criteria=u2 ~= 0  SaturateOnIntegerOverflow=off  InputSameDT=off
  Switch1 : Switch  Commented=on  Criteria=u2 ~= 0  SaturateOnIntegerOverflow=off  InputSameDT=off
  Switch4 : Switch  Commented=on  Criteria=u2 ~= 0  SaturateOnIntegerOverflow=off  InputSameDT=off
  Wind Turbine State Machine : Stateflow chart  TreatAsAtomicUnit=on
  T_g(t) : Outport
  β(t) : Outport  Port=2
  T_brake : Outport  Port=3
  orientation_sp : Outport  Port=4
  tag scope: CtrlState=global, logOpMode=global, logOrientationSpt=global, logPthSpt=global, logTBrake=global, logTGen=global
  wires:
  P_set(t)/1 -> Power controller/3(P_set(t))
  ω_g(t)/1 -> Power controller/4(ω_g(t))
  estop/1 -> Wind Turbine State Machine/4(estop)
  enable/1 -> Wind Turbine State Machine/3(enable)
  Wind Turbine State Machine/1(op_mode) -> [CtrlState], Compare To Constant10/1, Compare To Constant6/1, Compare To Constant4/1, Compare To Constant9/1, Compare To Constant3/1, Compare To Constant5/1, Compare To Constant/1, [logOpMode], Operational mode/1  "OpMode"
  Compare To Constant/1 -> Switch/2
  Switch/1 -> Switch3/3
  Constant1/1 -> Switch/1
  Constant/1 -> Switch/3
  Power controller/2(β(t)) -> Switch2/3  "β(t)"
  OR1/1 -> Switch2/2
  Compare To Constant3/1 -> OR1/1
  Compare To Constant4/1 -> OR1/3
  Compare To Constant5/1 -> OR1/2
  Constant4/1 -> "     "/1(deg)
  "     "/1(rad) -> Switch2/1  "pitch_parked"
  Switch2/1 -> [logPthSpt], β(t)/1  "PitchSpt"
  Compare To Constant6/1 -> OR2/1
  Exp/1 -> ?
  Gain/1 -> Exp/1
  Switch3/1 -> [logTBrake], T_brake/1  "Tbrake"
  Constant3/1 -> Switch3/1
  [rot_speed_sp] -> Wind Turbine State Machine/5(rot_speed_sp)
  [ctrl_mode] -> Wind Turbine State Machine/6(ctrl_mode)
  From3/1 -> Compare To Constant8/1
  des_orientation_sp/1 -> MATLAB Function/1(u)  "orientation_sp_SC"
  ctrl_mode/1 -> Power controller/5(ctrl_mode)
  Saturation/1 -> T_g(t)/1, [logTGen]  "Tgen"
  MATLAB Function/1(y) -> IC/1  "orientation_sp"
  Switch1/1 -> Switch4/3
  Compare To Constant2/1 -> OR/2
  Compare To Constant7/1 -> Switch4/2
  ? -> Switch1/3  "T_g(t)"
  OR/1 -> Switch1/2
  ? -> Compare To Constant7/1
  Compare To Constant1/1 -> OR/1
  ? -> Compare To Constant2/1
  Switch4/1 -> ?
  Constant5/1 -> Switch4/1
  Constant2/1 -> Switch1/1
  ? -> Compare To Constant1/1
  Constant6/1 -> Switch5/1
  Power controller/1(T_g(t)) -> Switch5/3  "T_g(t)"
  ws(t)/1 -> Moving Average/1, Power controller/1(ws(t))
  ω(t)/1 -> Wind Turbine State Machine/2(rot_speed), Power controller/2(ω(t))
  Switch5/1 -> Saturation/1
  Compare To Constant9/1 -> Switch5/2
  Moving Average/1 -> Wind Turbine State Machine/1(ws)
  Compare To Constant10/1 -> OR2/2
  OR2/1 -> Switch3/2
  IC/1 -> [logOrientationSpt], orientation_sp/1

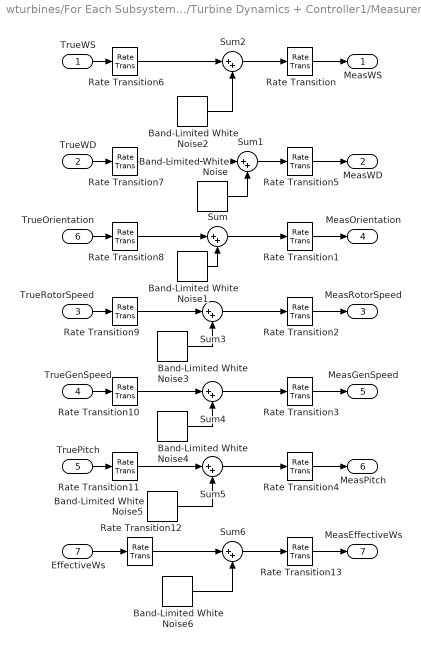
== system wturbines/For Each Subsystem/Turbine Dynamics + Controller1/Measurements ==
  TrueWS : Inport
  TrueWD : Inport  Port=2
  TrueRotorSpeed : Inport  Port=3
  TrueGenSpeed : Inport  Port=4
  TruePitch : Inport  Port=5
  TrueOrientation : Inport  Port=6
  EffectiveWs : Inport  Port=7
  Band-Limited White Noise : simulink/Sources/Band-Limited White Noise  Cov=[.5]  Ts=0.1  seed=[23341]
  Band-Limited White Noise1 : simulink/Sources/Band-Limited White Noise  Cov=[0.1]  Ts=0.1  seed=[23341]
  Band-Limited White Noise2 : simulink/Sources/Band-Limited White Noise  Cov=[0.01]  Ts=0.1  seed=[23341]
  Band-Limited White Noise3 : simulink/Sources/Band-Limited White Noise  Cov=[0.0001]  Ts=0.1  seed=[23341]
  Band-Limited White Noise4 : simulink/Sources/Band-Limited White Noise  Cov=[.001]  Ts=0.1  seed=[23341]
  Band-Limited White Noise5 : simulink/Sources/Band-Limited White Noise  Cov=[0.01]  Ts=0.1  seed=[23341]
  Band-Limited White Noise6 : simulink/Sources/Band-Limited White Noise  Cov=[0.1]  Ts=0.1  seed=[23341]
  Rate Transition{,1..13} (14 alike) : RateTransition
  Sum{,1..6} (7 alike) : Sum  Inputs=|++
  MeasWS : Outport
  MeasWD : Outport  Port=2
  MeasRotorSpeed : Outport  Port=3
  MeasOrientation : Outport  Port=4
  MeasGenSpeed : Outport  Port=5
  MeasPitch : Outport  Port=6
  MeasEffectiveWs : Outport  Port=7
  wires:
  TrueWS/1 -> Rate Transition6/1
  TrueWD/1 -> Rate Transition7/1
  TrueOrientation/1 -> Rate Transition8/1
  TrueRotorSpeed/1 -> Rate Transition9/1
  TruePitch/1 -> Rate Transition11/1
  TrueGenSpeed/1 -> Rate Transition10/1
  Sum1/1 -> Rate Transition5/1
  Sum/1 -> Rate Transition1/1
  Band-Limited White Noise/1 -> Sum1/2
  Band-Limited White Noise1/1 -> Sum/2
  Rate Transition/1 -> MeasWS/1
  Rate Transition5/1 -> MeasWD/1
  Rate Transition1/1 -> MeasOrientation/1
  Rate Transition2/1 -> MeasRotorSpeed/1
  Rate Transition3/1 -> MeasGenSpeed/1
  Rate Transition4/1 -> MeasPitch/1
  Rate Transition6/1 -> Sum2/1
  Rate Transition7/1 -> Sum1/1
  Rate Transition8/1 -> Sum/1
  Rate Transition9/1 -> Sum3/1
  Rate Transition10/1 -> Sum4/1
  Rate Transition11/1 -> Sum5/1
  Rate Transition12/1 -> Sum6/1
  Rate Transition13/1 -> MeasEffectiveWs/1
  EffectiveWs/1 -> Rate Transition12/1
  Band-Limited White Noise2/1 -> Sum2/2
  Band-Limited White Noise3/1 -> Sum3/2
  Sum3/1 -> Rate Transition2/1
  Sum4/1 -> Rate Transition3/1
  Band-Limited White Noise4/1 -> Sum4/2
  Sum5/1 -> Rate Transition4/1
  Band-Limited White Noise5/1 -> Sum5/2
  Sum6/1 -> Rate Transition13/1
  Band-Limited White Noise6/1 -> Sum6/2
  Sum2/1 -> Rate Transition/1

== system wturbines/For Each Subsystem/Turbine Dynamics + Controller1/Subsystem ==
  WsEff : Inport
  Constant : Constant  Value=rated_power
  Constant3 : Constant  Value=3
  Constant4 : Constant  Value=1/2
  Constant5 : Constant  Value=air_density
  Constant6 : Constant  Value=pi
  Constant7 : Constant  Value=rotor_radius
  Constant8 : Constant  Value=Cp_opt
  Constant9 : Constant  Value=generator_eff
  Min : MinMax  Inputs=2
  Power : Math  Operator=pow
  Product1 : Product  Inputs=7
  Square : Math  Operator=square
  P_avail : Outport
  wires:
  Constant5/1 -> Product1/2
  Constant3/1 -> Power/2
  Constant7/1 -> Square/1
  Constant9/1 -> Product1/6
  Constant6/1 -> Product1/3
  Square/1 -> Product1/4
  Product1/1 -> Min/1
  WsEff/1 -> Power/1
  Constant4/1 -> Product1/1
  Constant8/1 -> Product1/5
  Power/1 -> Product1/7  "ws_dr(t)"
  Constant/1 -> Min/2
  Min/1 -> P_avail/1

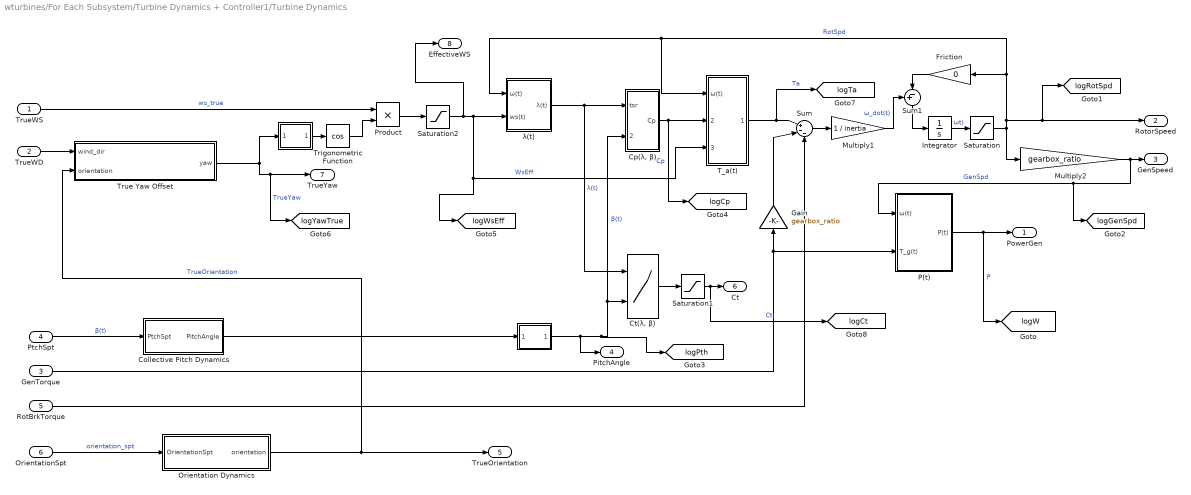
== system wturbines/For Each Subsystem/Turbine Dynamics + Controller1/Turbine Dynamics ==
  TrueWS : Inport
  TrueWD : Inport  Port=2
  GenTorque : Inport  Port=3
  PtchSpt : Inport  Port=4
  RotBrkTorque : Inport  Port=5
  OrientationSpt : Inport  Port=6
  "  " : Subsystem
  "     " : Subsystem
  Collective Pitch Dynamics : Subsystem
  "Cp(λ, β)" : Subsystem
  "Ct(λ, β)" : Lookup_n-D  BreakpointsForDimension1=tsr_vec  BreakpointsForDimension2=pitch_vec  Table=Ct_mat  InterpMethod=Cubic spline  ExtrapMethod=Clip  DiagnosticForOutOfRangeInput=Error  InternalRulePriority=Speed  RndMeth=Simplest
      settings: InputPortMap=u0,u1
  Friction : Gain  Gain=0
  Gain : Gain  Gain=gearbox_ratio
  Integrator : Integrator  LowerSaturationLimit=0
  Multiply1 : Gain  Gain=1 / inertia
  Multiply2 : Gain  Gain=gearbox_ratio
  Orientation Dynamics : Subsystem
  P(t) : Subsystem
  Product : Product
  Saturation : Saturate  UpperLimit=inf  LowerLimit=0
  Saturation1 : Saturate  UpperLimit=inf  LowerLimit=0
  Saturation2 : Saturate  UpperLimit=inf  LowerLimit=0
  Sum : Sum  Inputs=|+--
  Sum1 : Sum  Inputs=+-|
  T_a(t) : Subsystem
  Trigonometric Function : Trigonometry  Operator=cos
  True Yaw Offset : MATLAB Function  TreatAsAtomicUnit=on
  λ(t) : Subsystem
  PowerGen : Outport
  RotorSpeed : Outport  Port=2
  GenSpeed : Outport  Port=3
  PitchAngle : Outport  Port=4
  TrueOrientation : Outport  Port=5
  Ct : Outport  Port=6
  TrueYaw : Outport  Port=7
  EffectiveWS : Outport  Port=8
  tag scope: logCp=global, logCt=global, logGenSpd=global, logPth=global, logRotSpd=global, logTa=global, logW=global, logWsEff=global, logYawTrue=global
  wires:
  T_a(t)/1(T_a(t)) -> [logTa], Sum/1  "Ta"
  λ(t)/1(λ(t)) -> "Ct(λ, β)"/1, "Cp(λ, β)"/1(tsr)  "λ(t)"
  Multiply1/1 -> Sum1/1  "ω_dot(t)"
  Integrator/1 -> Saturation/1  "ωt)"
  Product/1 -> Saturation2/1
  "Cp(λ, β)"/1(Cp) -> T_a(t)/2(Cp(t)), [logCp]  "Cp"
  Sum/1 -> Multiply1/1
  RotBrkTorque/1 -> Sum/3
  P(t)/1(P(t)) -> [logW], PowerGen/1  "P"
  PtchSpt/1 -> Collective Pitch Dynamics/1(PtchSpt)  "β(t)"
  TrueWS/1 -> Product/1  "ws_true"
  Trigonometric Function/1 -> Product/2
  True Yaw Offset/1(yaw) -> [logYawTrue], TrueYaw/1, "     "/1(deg)  "TrueYaw"
  TrueWD/1 -> True Yaw Offset/1(wind_dir)
  "Ct(λ, β)"/1 -> Saturation1/1
  Multiply2/1 -> [logGenSpd], P(t)/1(ω(t)), GenSpeed/1  "GenSpd"
  Collective Pitch Dynamics/1(PitchAngle) -> "  "/1(rad)
  "  "/1(deg) -> PitchAngle/1, [logPth], "Ct(λ, β)"/2, "Cp(λ, β)"/2(pitch)  "β(t)"
  OrientationSpt/1 -> Orientation Dynamics/1(OrientationSpt)  "orientation_spt"
  Orientation Dynamics/1(orientation) -> TrueOrientation/1, True Yaw Offset/2(orientation)  "TrueOrientation"
  Saturation/1 -> [logRotSpd], RotorSpeed/1, Friction/1, λ(t)/1(ω(t)), T_a(t)/1(ω(t)), Multiply2/1  "RotSpd"
  Saturation1/1 -> [logCt], Ct/1  "Ct"
  "     "/1(rad) -> Trigonometric Function/1
  Saturation2/1 -> EffectiveWS/1, T_a(t)/3(ws(t)), [logWsEff], λ(t)/2(ws(t))  "WsEff"
  GenTorque/1 -> Gain/1, P(t)/2(T_g(t))
  Gain/1 -> Sum/2
  Friction/1 -> Sum1/2
  Sum1/1 -> Integrator/1

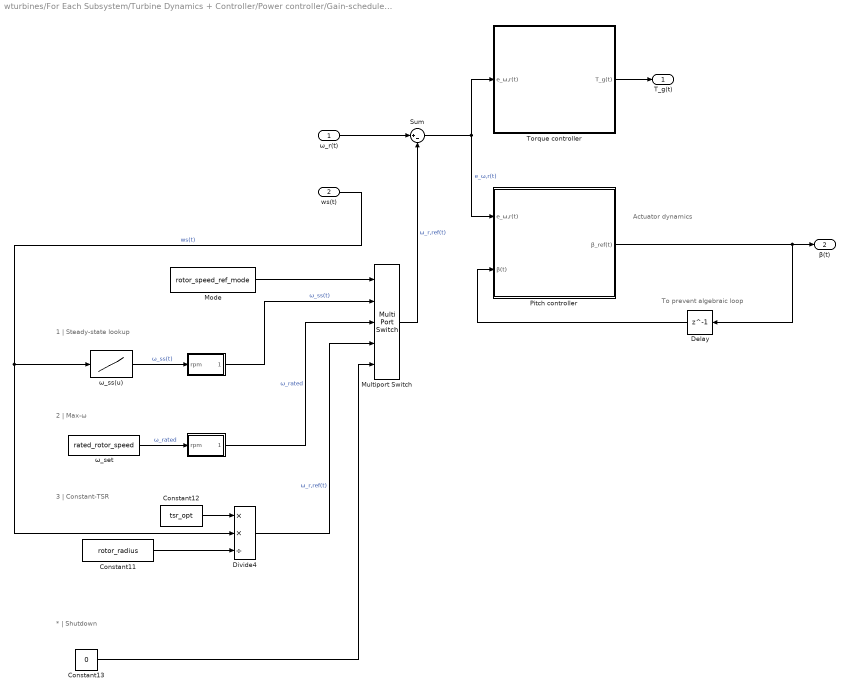
== system wturbines/For Each Subsystem/Turbine Dynamics + Controller/Power controller/Gain-scheduled H∞ control  ==
  note: 1 | Steady-state lookup
  note: * | Shutdown
  note: 2 | Max-ω
  note: 3 | Constant-TSR
  note: Actuator dynamics
  note: To prevent algebraic loop
  ω_r(t) : Inport
  ws(t) : Inport  Port=2
  " " : Subsystem
  "  " : Subsystem
  Constant11 : Constant  Value=rotor_radius
  Constant12 : Constant  Value=tsr_opt
  Constant13 : Constant  Value=0
  Delay : Delay  DelayLength=1
  Divide4 : Product  Inputs=**/
  Mode : Constant  Value=rotor_speed_ref_mode
  Multiport Switch : MultiPortSwitch  DataPortForDefault=Additional data port  DiagnosticForDefault=None  SaturateOnIntegerOverflow=off  InputSameDT=off
  Pitch controller : Subsystem
  Sum : Sum  Inputs=|+-
  Torque controller : Subsystem
  ω_set : Constant  Value=rated_rotor_speed
  ω_ss(u) : Lookup_n-D  NumberOfTableDimensions=1  BreakpointsForDimension1=u_rotor_speed_all  Table=rotor_speed_all  InternalRulePriority=Speed  RndMeth=Simplest
  T_g(t) : Outport
  β(t) : Outport  Port=2
  wires:
  "  "/1(rad/s) -> Multiport Switch/3  "ω_rated"
  " "/1(rad/s) -> Multiport Switch/2  "ω_ss(t)"
  ω_ss(u)/1 -> " "/1(rpm)  "ω_ss(t)"
  ws(t)/1 -> Divide4/2, ω_ss(u)/1  "ws(t)"
  ω_r(t)/1 -> Sum/1
  Multiport Switch/1 -> Sum/2  "ω_r,ref(t)"
  ω_set/1 -> "  "/1(rpm)  "ω_rated"
  Constant13/1 -> Multiport Switch/5
  Divide4/1 -> Multiport Switch/4  "ω_r,ref(t)"
  Constant11/1 -> Divide4/3
  Mode/1 -> Multiport Switch/1
  Constant12/1 -> Divide4/1
  Sum/1 -> Torque controller/1(e_ω,r(t)), Pitch controller/1(e_ω,r(t))  "e_ω,r(t)"
  Delay/1 -> Pitch controller/2(β(t))
  Pitch controller/1(β_ref(t)) -> β(t)/1, Delay/1
  Torque controller/1(T_g(t)) -> T_g(t)/1

== system wturbines/For Each Subsystem/Turbine Dynamics + Controller/Power controller/Kω2 controller ==
  ω(t) : Inport
  ws(t) : Inport  Port=2
  Pitch controller : Subsystem
  Torque controller : Subsystem
  T_g(t) : Outport
  β(t) : Outport  Port=2
  wires:
  ws(t)/1 -> Pitch controller/1(ws(t))
  ω(t)/1 -> Torque controller/1(ω(t)), Pitch controller/2(ω(t))
  Pitch controller/1(β(t)) -> β(t)/1
  Torque controller/1(T_g(t)) -> T_g(t)/1

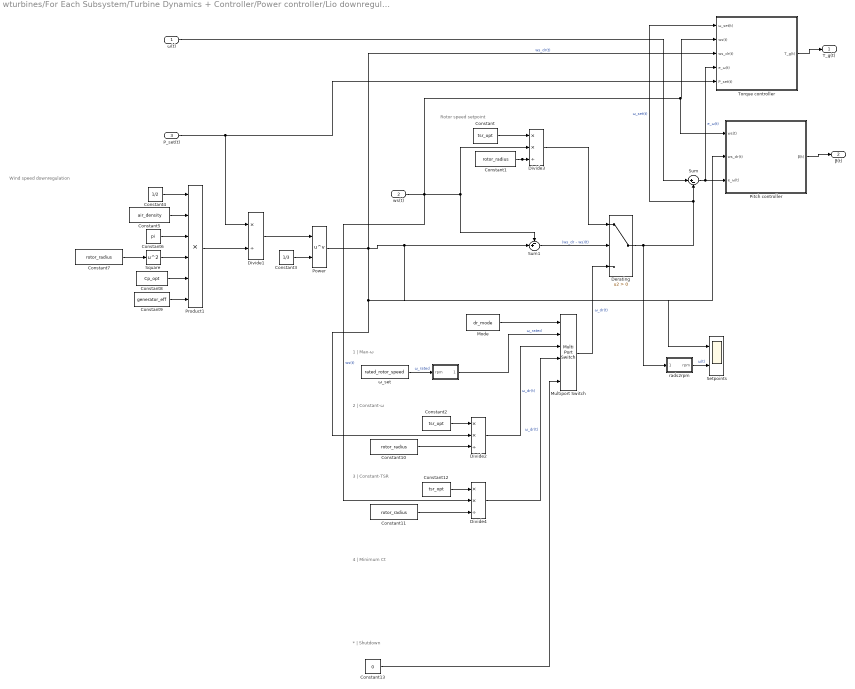
== system wturbines/For Each Subsystem/Turbine Dynamics + Controller/Power controller/Lio downregulation ==
  note: * | Shutdown
  note: 4 | Minimum Ct
  note: 3 | Constant-TSR
  note: 2 | Constant-ω
  note: Rotor speed setpoint
  note: Wind speed downregulation
  note: 1 | Max-ω
  ω(t) : Inport
  ws(t) : Inport  Port=2
  P_set(t) : Inport  Port=3
  "  " : Subsystem
  Constant : Constant  Value=tsr_opt
  Constant{1,7,10..11} (4 alike) : Constant  Value=rotor_radius
  Constant12 : Constant  Value=tsr_opt
  Constant13 : Constant  Value=0
  Constant2 : Constant  Value=tsr_opt
  Constant3 : Constant  Value=1/3
  Constant4 : Constant  Value=1/2
  Constant5 : Constant  Value=air_density
  Constant6 : Constant  Value=pi
  Constant8 : Constant  Value=Cp_opt
  Constant9 : Constant  Value=generator_eff
  Derating : Switch  Criteria=u2 > Threshold  SaturateOnIntegerOverflow=off  InputSameDT=off
  Divide1 : Product  Inputs=*/
  Divide2 : Product  Inputs=**/
  Divide3 : Product  Inputs=**/
  Divide4 : Product  Inputs=**/
  Mode : Constant  Value=dr_mode
  Multiport Switch : MultiPortSwitch  Inputs=4  DataPortForDefault=Additional data port  DiagnosticForDefault=None  SaturateOnIntegerOverflow=off  InputSameDT=off
  Pitch controller : Subsystem
  Power : Math  Operator=pow
  Product1 : Product  Inputs=6
  Setpoints : Scope  NumInputPorts=2
  Square : Math  Operator=square
  Sum : Sum  Inputs=|+-
  Sum1 : Sum  Inputs=-+|
  Torque controller : Subsystem
  rads2rpm : Subsystem
  ω_set : Constant  Value=rated_rotor_speed
  T_g(t) : Outport
  β(t) : Outport  Port=2
  wires:
  "  "/1(rad/s) -> Multiport Switch/2  "ω_rated"
  rads2rpm/1(rpm) -> Setpoints/2  "ω(t)"
  Constant13/1 -> Multiport Switch/6
  Divide4/1 -> Multiport Switch/4  "ω_dr(t)"
  Constant12/1 -> Divide4/1
  Constant11/1 -> Divide4/3
  Mode/1 -> Multiport Switch/1
  Multiport Switch/1 -> Derating/3  "ω_dr(t)"
  Constant10/1 -> Divide2/3
  Constant2/1 -> Divide2/1
  Divide2/1 -> Multiport Switch/3  "ω_dr(t)"
  ω_set/1 -> "  "/1(rpm)  "ω_rated"
  ω(t)/1 -> Sum/1
  Constant9/1 -> Product1/6
  Constant8/1 -> Product1/5
  Square/1 -> Product1/4
  Constant7/1 -> Square/1
  Constant6/1 -> Product1/3
  Constant5/1 -> Product1/2
  Constant4/1 -> Product1/1
  Product1/1 -> Divide1/2
  Divide1/1 -> Power/1
  P_set(t)/1 -> Divide1/1, Torque controller/5(P_set(t))
  Constant3/1 -> Power/2
  ws(t)/1 -> Sum1/1, Divide3/2, Torque controller/2(ws(t)), Pitch controller/1(ws(t)), Divide4/2  "ws(t)"
  Power/1 -> Torque controller/3(ws_dr(t)), Pitch controller/2(ws_dr(t)), Divide2/2, Sum1/2, Setpoints/1  "ws_dr(t)"
  Sum1/1 -> Derating/2  "(ws_dr - ws)(t)"
  Constant/1 -> Divide3/1
  Constant1/1 -> Divide3/3
  Divide3/1 -> Derating/1
  Sum/1 -> Pitch controller/3(e_ω(t)), Torque controller/4(e_ω(t))  "e_ω(t)"
  Derating/1 -> Sum/2, Torque controller/1(ω_set(t)), rads2rpm/1(rad/s)  "ω_set(t)"
  Pitch controller/1(β(t)) -> β(t)/1
  Torque controller/1(T_g(t)) -> T_g(t)/1

== system wturbines/For Each Subsystem/Turbine Dynamics + Controller/Power controller/ROSCO ==
  note: Pitch saturation
  note: Setpoint smoother
  ω_r(t) : Inport
  ws(t) : Inport  Port=2
  ω_g(t) : Inport  Port=3
  Pitch controller : Subsystem
  Torque controller : Subsystem
  T_g(t) : Outport
  β(t) : Outport  Port=2
  wires:
  ? -> Pitch controller/2(Δω_g(t)), Torque controller/3(Δω_g(t))  "Δω_g(t)"
  Pitch controller/1(β(t)) -> β(t)/1, Torque controller/4(β(t))
  Torque controller/1(T_g(t)) -> T_g(t)/1

== system wturbines/For Each Subsystem/Turbine Dynamics + Controller/Subsystem/Yaw controller ==
  note: Here we assume a simple model for now:
      | - Orientation set-point is instantly met
      | - We assume we can measure the orientation perfectly
  orientation_set(t) : Inport
  orientation(t) : Outport
  wires:
  orientation_set(t)/1 -> orientation(t)/1

== system wturbines/For Each Subsystem/Turbine Dynamics + Controller1/Control logic/      ==
  deg : Inport
  Degrees to Radians : simulink_extras/Transformations/Degrees to Radians
  rad : Outport
  wires:
  deg/1 -> Degrees to Radians/1
  Degrees to Radians/1 -> rad/1
